simulink model "RC1_Simulink_Demo"  (R2025a)
settings: Solver=ode45  StartTime=0.0  StopTime=240  MaxStep=1  RelTol=1e-3
settings Model: Creator=13175  LastModifiedBy=13175

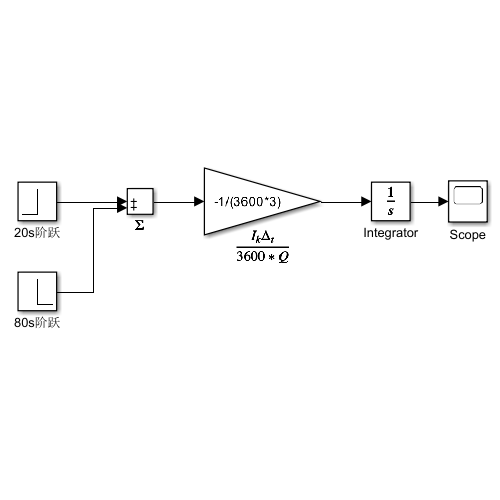
[thumbnail: Simulink's stored preview of the top-level diagram]
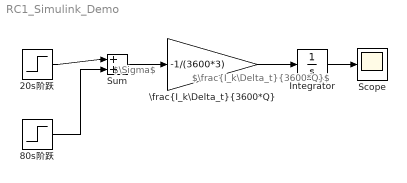
== system RC1_Simulink_Demo ==
  note: $\Sigma$
  note: $\frac{I_k\Delta_t}{3600*Q}$
  20s阶跃 : Step  Time=20  After=2  SampleTime=1
  80s阶跃 : Step  Time=80  After=-2  SampleTime=1
  Integrator : Integrator  InitialCondition=0.8
  Scope : Scope
      settings: ActiveDisplayYMinimum=0.78750000000000064  ActiveDisplayYMaximum=0.80138888888888893
  Sum : Sum  Inputs=|++
  "\\frac{I_k\\Delta_t}{3600*Q}" : Gain  Gain=-1/(3600*3)
  wires:
  20s阶跃/1 -> Sum/1
  80s阶跃/1 -> Sum/2
  Sum/1 -> "\\frac{I_k\\Delta_t}{3600*Q}"/1
  "\\frac{I_k\\Delta_t}{3600*Q}"/1 -> Integrator/1
  Integrator/1 -> Scope/1
